simulink model "TB14_StageC_Regulated"  (R2025a)
settings: Solver=FixedStepDiscrete  StartTime=0  StopTime=TB.t_end  FixedStep=TB.dt  RelTol=1e-3
InitFcn:
  | % 모델과 같은 폴더의 초기화 스크립트를 실행해 P(설계 파라미터)와 TB(시험 조건)를 만든다.
  | run(fullfile(fileparts(get_param(bdroot, 'FileName')), 'TB14_init.m'));
values from neighbouring files (symbols this model uses):
  TB = struct()    [TB14_init.m]    (also in probe_TB14_solver.m = evalin('base', 'TB'); run_TB14.m = evalin('base', 'TB'))
libraries: fl_lib x59, nesl_utility x27
(part 1 of 2)
settings Model: Creator=hj000  LastModifiedBy=hj000
settings DataIOCC: SaveOutput=off  SignalLogging=off  SaveTime=off

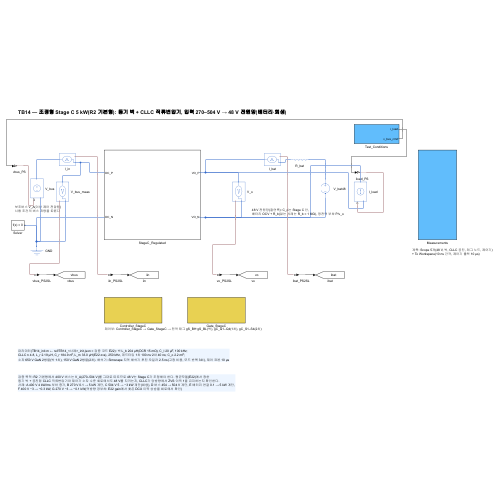
[thumbnail: Simulink's stored preview of the top-level diagram]
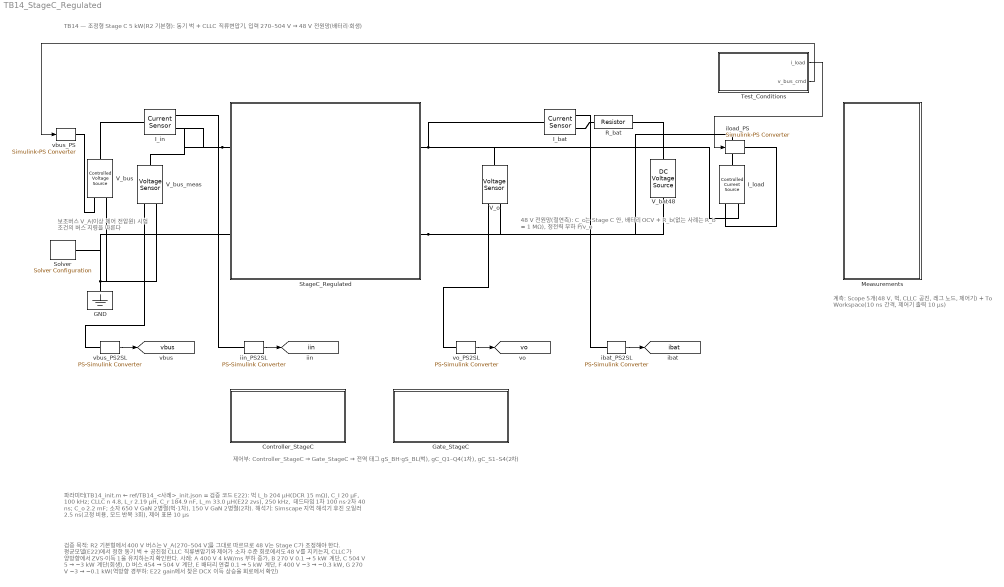
== system TB14_StageC_Regulated ==
  note: TB14 — 조정형 Stage C 5 kW(R2 기본형): 동기 벅 + CLLC 직류변압기, 입력 270–504 V → 48 V 전원망(배터리·회생)
  note: 보조버스 V_A(이상 제어 전압원)
      | 시험 조건의 버스 지령을 따른다
  note: 48 V 전원망(절연측): C_o는 Stage C 안,
      | 배터리 OCV + R_b(없는 사례는 R_b = 1 MΩ), 정전력 부하 P/v_o
  note: 제어부: Controller_StageC → Gate_StageC → 전역 태그 gS_BH·gS_BL(벅), gC_Q1–Q4(1차), gC_S1–S4(2차)
  note: 계측: Scope 5개(48 V, 벅, CLLC 공진, 레그 노드, 제어기)
      | + To Workspace(10 ns 간격, 제어기 출력 10 µs)
  note: 파라미터(TB14_init.m ← ref/TB14_<사례>_init.json = 검증 코드 E22): 벅 L_b 204 µH(DCR 15 mΩ), C_I 20 µF, 100 kHz;
      | CLLC n 4.8, L_r 2.19 µH, C_r 184.9 nF, L_m 33.0 µH(E22 zvs), 250 kHz, 데드타임 1차 100 ns·2차 40 ns; C_o 2.2 mF;
      | 소자 650 V GaN 2병렬(벅·1차), 150 V GaN 2병렬(2차). 해석기: Simscape 지역 해석기 후진 오일러 2.5 ns(고정 비용, 모드 반복 3회), 제어 표본 10 µs
  note: 검증 목적: R2 기본형에서 400 V 버스는 V_A(270–504 V)를 그대로 따르므로 48 V는 Stage C가 조정해야 한다. 평균모델(E22)에서 정한
      | 동기 벅 + 공진점 CLLC 직류변압기와 제어가 소자 수준 회로에서도 48 V를 지키는지, CLLC가 양방향에서 ZVS·이득 1을 유지하는지 확인한다.
      | 사례: A 400 V 4 kW/ms 부하 증가, B 270 V 0.1 → 5 kW 계단, C 504 V 5 → −3 kW 계단(회생), D 버스 454 → 504 V 계단, E 배터리 연결 0.1 → 5 kW 계단,
      | F 400 V −3 → −0.3 kW, G 270 V −3 → −0.1 kW(역방향 경부하: E22 gain에서 찾은 DCX 이득 상승을 회로에서 확인)
  Controller_StageC : Subsystem
  GND : fl_lib/Electrical/Electrical Elements/Electrical Reference
  Gate_StageC : Subsystem
  I_bat : fl_lib/Electrical/Electrical Sensors/Current Sensor
  I_in : fl_lib/Electrical/Electrical Sensors/Current Sensor
  I_load : fl_lib/Electrical/Electrical Sources/Controlled Current Source
  Measurements : Subsystem
  R_bat : fl_lib/Electrical/Electrical Elements/Resistor  R=TB.Rbat Ohm  i_specify=off  i_priority=None  i=0 A  i_nominal_specify=off  i_nominal_value=1  i_nominal_unit=A  v_specify=off  v_priority=None  v=0 V  v_nominal_specify=off  v_nominal_value=1  v_nominal_unit=V
  Solver : nesl_utility/Solver Configuration  PhysicalDomain=network_engine_domain  SubClassName=solver  LeftPortType=input  RightPortType=generic  Tones=[]  Harmonics=[]  SimulateNoise=off  Profile=off  UseLocalSampling=off  EnableSwitchedLinearOptims=on  FrequencyDomain=off  UseCCode=off  RelTol=0.001  AbsTol=0.001  MinStep=1e-09  ToWorkspace=off  RevertToSquareIcSolve=off  NumHomotopyIterations=100  PhasorMode=off  PhasorModeNumHarmonics=1  ConsistencySolver=NEWTON_XTOL_AFTER_FTOL  IndexReductionMethod=DerivativeReplacement  DoDC=off  ResidualTolerance=1e-9  ConsistencyTolSource=GLOBAL  ConsistencyAbsTol=0.001  ConsistencyRelTol=0.001  ConsistencyTolFactor=0.001  UseLocalSolver=on  LocalSolverChoice=NE_BACKWARD_EULER_ADVANCER  ResolveIndetEquations=on  FunctionEvalNumThread=1  LocalSolverSampleTime=TB.dt  DoFixedCost=on  MaxNonlinIter=3  MaxModeIter=2  ComputeImpulses=off  ImpulseIterations=2  LinearAlgebra=auto  LinearAlgebraNumThread=0  EquationFormulation=NE_TIME_EF  DelaysMemoryBudget=1024  AutomaticFiltering=on  FilteringTimeConstant=0.001  PartitionStorageMethod=AS_NEEDED  PartitionMemoryBudget=1024  PartitionMethod=ROBUST  MultibodyUseLocalSolver=off  MultibodyLocalSolverChoice=ODE1  MultibodyLocalSolverSampleTime=0.001
  StageC_Regulated : Subsystem
  Test_Conditions : Subsystem
  V_bat48 : fl_lib/Electrical/Electrical Sources/DC Voltage Source  v0=TB.OCV V
  V_bus : fl_lib/Electrical/Electrical Sources/Controlled Voltage Source
  V_bus_meas : fl_lib/Electrical/Electrical Sensors/Voltage Sensor
  V_o : fl_lib/Electrical/Electrical Sensors/Voltage Sensor
  ibat_PS2SL : nesl_utility/PS-Simulink Converter  PhysicalDomain=network_engine_domain  SubClassName=ps_output  LeftPortType=input  RightPortType=output  PseudoPeriodic=off  Frequencies=[]  VectorFormat=inherit  Unit=inherit  AffineConversion=off
  iin_PS2SL : nesl_utility/PS-Simulink Converter  PhysicalDomain=network_engine_domain  SubClassName=ps_output  LeftPortType=input  RightPortType=output  PseudoPeriodic=off  Frequencies=[]  VectorFormat=inherit  Unit=inherit  AffineConversion=off
  iload_PS : nesl_utility/Simulink-PS Converter  PhysicalDomain=network_engine_domain  SubClassName=ps_input  LeftPortType=input  RightPortType=output  PseudoPeriodic=off  Frequencies=[]  NoiseDistribution=none  NoiseParameters=[]  Unit=1  AffineConversion=off  FilteringAndDerivatives=provide  SimscapeFilterOrder=1  InputFilterTimeConstant=0.001  UdotUserProvided=0
  vbus_PS : nesl_utility/Simulink-PS Converter  PhysicalDomain=network_engine_domain  SubClassName=ps_input  LeftPortType=input  RightPortType=output  PseudoPeriodic=off  Frequencies=[]  NoiseDistribution=none  NoiseParameters=[]  Unit=1  AffineConversion=off  FilteringAndDerivatives=provide  SimscapeFilterOrder=1  InputFilterTimeConstant=0.001  UdotUserProvided=0
  vbus_PS2SL : nesl_utility/PS-Simulink Converter  PhysicalDomain=network_engine_domain  SubClassName=ps_output  LeftPortType=input  RightPortType=output  PseudoPeriodic=off  Frequencies=[]  VectorFormat=inherit  Unit=inherit  AffineConversion=off
  vo_PS2SL : nesl_utility/PS-Simulink Converter  PhysicalDomain=network_engine_domain  SubClassName=ps_output  LeftPortType=input  RightPortType=output  PseudoPeriodic=off  Frequencies=[]  VectorFormat=inherit  Unit=inherit  AffineConversion=off
  tag scope: ibat=global, iin=global, vbus=global, vo=global
  wires:
  vbus_PS2SL/1 -> [vbus]
  iin_PS2SL/1 -> [iin]
  vo_PS2SL/1 -> [vo]
  ibat_PS2SL/1 -> [ibat]
  Test_Conditions/1(i_load) -> iload_PS/1
  Test_Conditions/2(v_bus_cmd) -> vbus_PS/1
  connections:
  Solver/RConn1 -- V_bus/RConn2 -- StageC_Regulated/LConn2 -- GND/LConn1 -- V_bus_meas/RConn2
  vbus_PS/RConn1 -- V_bus/RConn1
  V_bus/LConn1 -- I_in/LConn1
  StageC_Regulated/LConn1 -- I_in/RConn2 -- V_bus_meas/LConn1
  V_o/LConn1 -- I_bat/LConn1 -- StageC_Regulated/RConn1 -- I_load/RConn2
  V_o/RConn2 -- V_bat48/RConn1 -- StageC_Regulated/RConn2 -- I_load/LConn1
  I_bat/RConn2 -- R_bat/LConn1
  R_bat/RConn1 -- V_bat48/LConn1
  iload_PS/RConn1 -- I_load/RConn1
  V_bus_meas/RConn1 -- vbus_PS2SL/LConn1
  I_in/RConn1 -- iin_PS2SL/LConn1
  V_o/RConn1 -- vo_PS2SL/LConn1
  I_bat/RConn1 -- ibat_PS2SL/LConn1

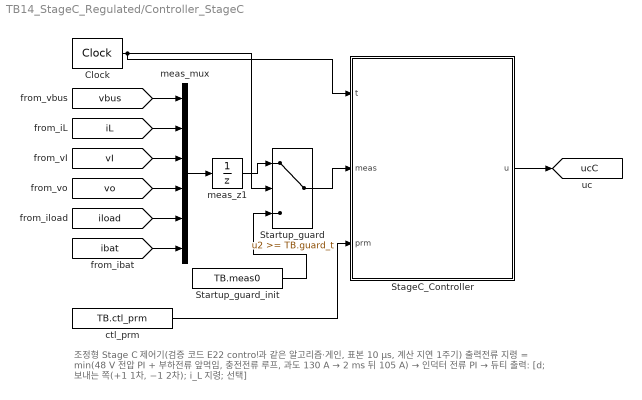
== system TB14_StageC_Regulated/Controller_StageC ==
  note: 조정형 Stage C 제어기(검증 코드 E22 control과 같은 알고리즘·게인, 표본 10 µs, 계산 지연 1주기)
      | 출력전류 지령 = min(48 V 전압 PI + 부하전류 앞먹임, 충전전류 루프, 과도 130 A → 2 ms 뒤 105 A) → 인덕터 전류 PI → 듀티
      | 출력: [d; 보내는 쪽(+1 1차, −1 2차); i_L 지령; 선택]
  Clock : DigitalClock  SampleTime=TB.dt
  StageC_Controller : MATLAB Function  TreatAsAtomicUnit=on
  Startup_guard : Switch  Threshold=TB.guard_t  SaturateOnIntegerOverflow=off  InputSameDT=off
  Startup_guard_init : Constant  Value=TB.meas0
  ctl_prm : Constant  Value=TB.ctl_prm
  meas_mux : Mux  Inputs=6
  meas_z1 : UnitDelay  InitialCondition=TB.meas0  SampleTime=TB.dt  HasFrameUpgradeWarning=on
  tag scope: ucC=global
  wires:
  [vbus] -> meas_mux/1
  [iL] -> meas_mux/2
  [vI] -> meas_mux/3
  [vo] -> meas_mux/4
  [iload] -> meas_mux/5
  [ibat] -> meas_mux/6
  meas_mux/1 -> meas_z1/1
  Startup_guard_init/1 -> Startup_guard/3
  meas_z1/1 -> Startup_guard/1
  Clock/1 -> Startup_guard/2, StageC_Controller/1(t)
  Startup_guard/1 -> StageC_Controller/2(meas)
  ctl_prm/1 -> StageC_Controller/3(prm)
  StageC_Controller/1(u) -> [ucC]

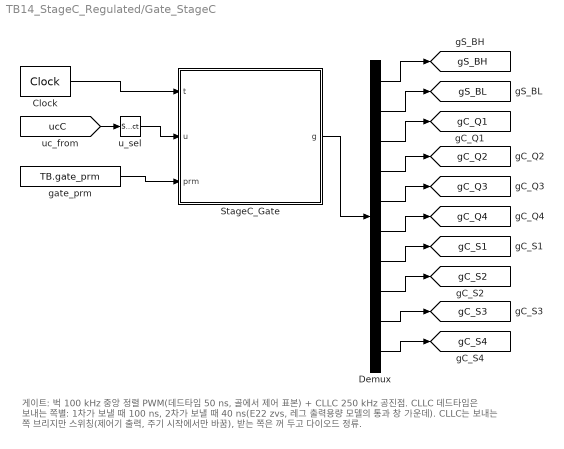
== system TB14_StageC_Regulated/Gate_StageC ==
  note: 게이트: 벅 100 kHz 중앙 정렬 PWM(데드타임 50 ns, 골에서 제어 표본) + CLLC 250 kHz 공진점.
      | CLLC 데드타임은 보내는 쪽별: 1차가 보낼 때 100 ns, 2차가 보낼 때 40 ns(E22 zvs, 레그 출력용량 모델의 통과 창 가운데).
      | CLLC는 보내는 쪽 브리지만 스위칭(제어기 출력, 주기 시작에서만 바꿈), 받는 쪽은 꺼 두고 다이오드 정류.
  Clock : DigitalClock  SampleTime=TB.dt
  Demux : Demux  Outputs=10
  StageC_Gate : MATLAB Function  TreatAsAtomicUnit=on
  gate_prm : Constant  Value=TB.gate_prm
  u_sel : Selector  InputPortWidth=4  IndexOptions=Index vector (dialog)  Indices=[1 2]  OutputSizes=1
  tag scope: gC_Q1=global, gC_Q2=global, gC_Q3=global, gC_Q4=global, gC_S1=global, gC_S2=global, gC_S3=global, gC_S4=global, gS_BH=global, gS_BL=global
  wires:
  [ucC] -> u_sel/1
  Clock/1 -> StageC_Gate/1(t)
  u_sel/1 -> StageC_Gate/2(u)
  gate_prm/1 -> StageC_Gate/3(prm)
  StageC_Gate/1(g) -> Demux/1
  Demux/1 -> [gS_BH]
  Demux/2 -> [gS_BL]
  Demux/3 -> [gC_Q1]
  Demux/4 -> [gC_Q2]
  Demux/5 -> [gC_Q3]
  Demux/6 -> [gC_Q4]
  Demux/7 -> [gC_S1]
  Demux/8 -> [gC_S2]
  Demux/9 -> [gC_S3]
  Demux/10 -> [gC_S4]

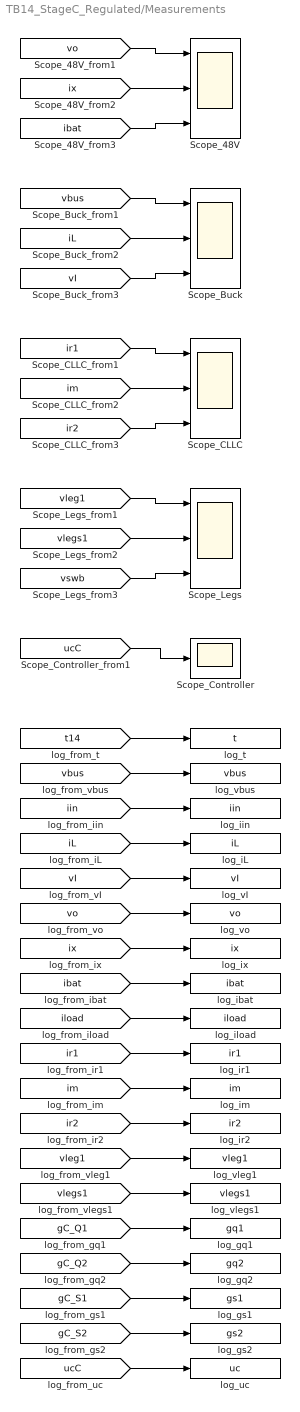
== system TB14_StageC_Regulated/Measurements ==
  Scope_48V : Scope  NumInputPorts=3
      settings: Title=Scope 48V
  Scope_Buck : Scope  NumInputPorts=3
      settings: Title=Scope Buck
  Scope_CLLC : Scope  NumInputPorts=3
      settings: Title=Scope CLLC
  Scope_Controller : Scope
      settings: Title=Scope Controller
  Scope_Legs : Scope  NumInputPorts=3
      settings: Title=Scope Legs
  log_gq1 : ToWorkspace  VariableName=gq1  SampleTime=-1
      settings: Decimation=4
  log_gq2 : ToWorkspace  VariableName=gq2  SampleTime=-1
      settings: Decimation=4
  log_gs1 : ToWorkspace  VariableName=gs1  SampleTime=-1
      settings: Decimation=4
  log_gs2 : ToWorkspace  VariableName=gs2  SampleTime=-1
      settings: Decimation=4
  log_iL : ToWorkspace  VariableName=iL  SampleTime=-1
      settings: Decimation=4
  log_ibat : ToWorkspace  VariableName=ibat  SampleTime=-1
      settings: Decimation=4
  log_iin : ToWorkspace  VariableName=iin  SampleTime=-1
      settings: Decimation=4
  log_iload : ToWorkspace  VariableName=iload  SampleTime=-1
      settings: Decimation=4
  log_im : ToWorkspace  VariableName=im  SampleTime=-1
      settings: Decimation=4
  log_ir1 : ToWorkspace  VariableName=ir1  SampleTime=-1
      settings: Decimation=4
  log_ir2 : ToWorkspace  VariableName=ir2  SampleTime=-1
      settings: Decimation=4
  log_ix : ToWorkspace  VariableName=ix  SampleTime=-1
      settings: Decimation=4
  log_t : ToWorkspace  VariableName=t  SampleTime=-1
      settings: Decimation=4
  log_uc : ToWorkspace  VariableName=uc  SampleTime=-1
      settings: Decimation=4000
  log_vI : ToWorkspace  VariableName=vI  SampleTime=-1
      settings: Decimation=4
  log_vbus : ToWorkspace  VariableName=vbus  SampleTime=-1
      settings: Decimation=4
  log_vleg1 : ToWorkspace  VariableName=vleg1  SampleTime=-1
      settings: Decimation=4
  log_vlegs1 : ToWorkspace  VariableName=vlegs1  SampleTime=-1
      settings: Decimation=4
  log_vo : ToWorkspace  VariableName=vo  SampleTime=-1
      settings: Decimation=4
  wires:
  [vo] -> Scope_48V/1
  [ix] -> Scope_48V/2
  [ibat] -> Scope_48V/3
  [vbus] -> Scope_Buck/1
  [iL] -> Scope_Buck/2
  [vI] -> Scope_Buck/3
  [ir1] -> Scope_CLLC/1
  [im] -> Scope_CLLC/2
  [ir2] -> Scope_CLLC/3
  [vleg1] -> Scope_Legs/1
  [vlegs1] -> Scope_Legs/2
  [vswb] -> Scope_Legs/3
  [ucC] -> Scope_Controller/1
  [t14] -> log_t/1
  [vbus] -> log_vbus/1
  [iin] -> log_iin/1
  [iL] -> log_iL/1
  [vI] -> log_vI/1
  [vo] -> log_vo/1
  [ix] -> log_ix/1
  [ibat] -> log_ibat/1
  [iload] -> log_iload/1
  [ir1] -> log_ir1/1
  [im] -> log_im/1
  [ir2] -> log_ir2/1
  [vleg1] -> log_vleg1/1
  [vlegs1] -> log_vlegs1/1
  [gC_Q1] -> log_gq1/1
  [gC_Q2] -> log_gq2/1
  [gC_S1] -> log_gs1/1
  [gC_S2] -> log_gs2/1
  [ucC] -> log_uc/1

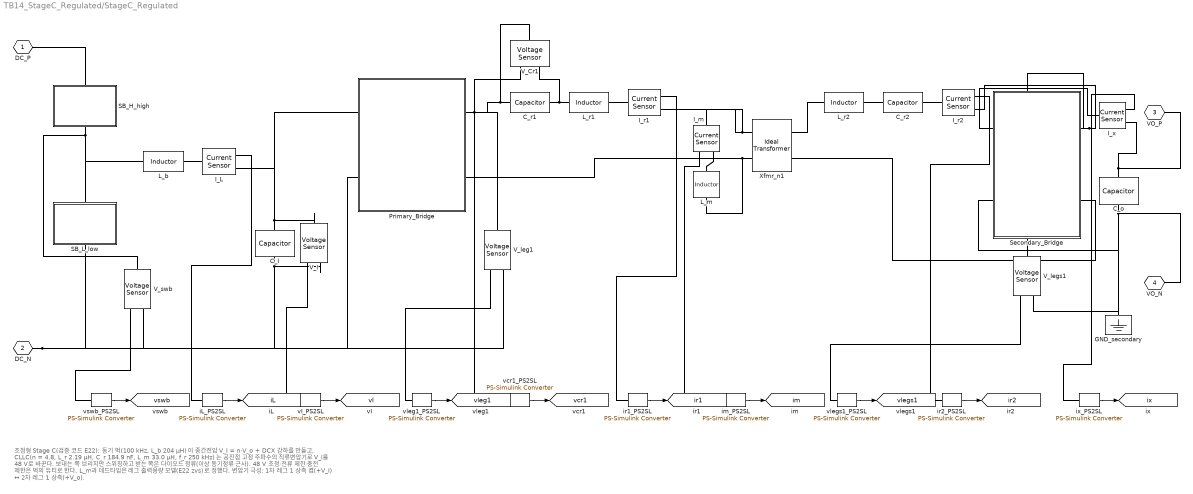
== system TB14_StageC_Regulated/StageC_Regulated ==
  note: 조정형 Stage C(검증 코드 E22): 동기 벅(100 kHz, L_b 204 µH)이 중간전압 V_I = n·V_o + DCX 강하를 만들고,
      | CLLC(n = 4.8, L_r 2.19 µH, C_r 184.9 nF, L_m 33.0 µH, f_r 250 kHz)는 공진점 고정 주파수의 직류변압기로 V_I를 48 V로 바꾼다.
      | 보내는 쪽 브리지만 스위칭하고 받는 쪽은 다이오드 정류(이상 동기정류 근사). 48 V 조정·전류 제한·충전 제한은 벅의 듀티로 한다.
      | L_m과 데드타임은 레그 출력용량 모델(E22 zvs)로 정했다. 변압기 극성: 1차 레그 1 상측 켬(+V_I) ↔ 2차 레그 1 상측(+V_o).
  C_I : fl_lib/Electrical/Electrical Elements/Capacitor  c=TB.C.CI F  r=1e-6 Ohm  g=0 1/Ohm  i_specify=off  i_priority=None  i=0 A  i_nominal_specify=off  i_nominal_value=1  i_nominal_unit=A  v_specify=off  v_priority=None  v=0 V  v_nominal_specify=off  v_nominal_value=1  v_nominal_unit=V  vc_specify=on  vc_priority=High  vc=TB.x0(2) V  vc_nominal_specify=off  vc_nominal_value=1  vc_nominal_unit=V
  C_o : fl_lib/Electrical/Electrical Elements/Capacitor  c=TB.C.Co F  r=1e-6 Ohm  g=0 1/Ohm  i_specify=off  i_priority=None  i=0 A  i_nominal_specify=off  i_nominal_value=1  i_nominal_unit=A  v_specify=off  v_priority=None  v=0 V  v_nominal_specify=off  v_nominal_value=1  v_nominal_unit=V  vc_specify=on  vc_priority=High  vc=TB.x0(3) V  vc_nominal_specify=off  vc_nominal_value=1  vc_nominal_unit=V
  C_r1 : fl_lib/Electrical/Electrical Elements/Capacitor  c=TB.C.Cr1 F  r=1e-6 Ohm  g=0 1/Ohm  i_specify=off  i_priority=None  i=0 A  i_nominal_specify=off  i_nominal_value=1  i_nominal_unit=A  v_specify=off  v_priority=None  v=0 V  v_nominal_specify=off  v_nominal_value=1  v_nominal_unit=V  vc_specify=on  vc_priority=High  vc=0 V  vc_nominal_specify=off  vc_nominal_value=1  vc_nominal_unit=V
  C_r2 : fl_lib/Electrical/Electrical Elements/Capacitor  c=TB.C.Cr2 F  r=1e-6 Ohm  g=0 1/Ohm  i_specify=off  i_priority=None  i=0 A  i_nominal_specify=off  i_nominal_value=1  i_nominal_unit=A  v_specify=off  v_priority=None  v=0 V  v_nominal_specify=off  v_nominal_value=1  v_nominal_unit=V  vc_specify=on  vc_priority=High  vc=0 V  vc_nominal_specify=off  vc_nominal_value=1  vc_nominal_unit=V
  GND_secondary : fl_lib/Electrical/Electrical Elements/Electrical Reference
  I_L : fl_lib/Electrical/Electrical Sensors/Current Sensor
  I_m : fl_lib/Electrical/Electrical Sensors/Current Sensor
  I_r1 : fl_lib/Electrical/Electrical Sensors/Current Sensor
  I_r2 : fl_lib/Electrical/Electrical Sensors/Current Sensor
  I_x : fl_lib/Electrical/Electrical Sensors/Current Sensor
  L_b : fl_lib/Electrical/Electrical Elements/Inductor  l=TB.C.L H  r=TB.C.RL Ohm  g=1e-9 1/Ohm  i_specify=off  i_priority=None  i=0 A  i_nominal_specify=off  i_nominal_value=1  i_nominal_unit=A  v_specify=off  v_priority=None  v=0 V  v_nominal_specify=off  v_nominal_value=1  v_nominal_unit=V  i_L_specify=on  i_L_priority=High  i_L=TB.x0(1) A  i_L_nominal_specify=off  i_L_nominal_value=1  i_L_nominal_unit=A
  L_m : fl_lib/Electrical/Electrical Elements/Inductor  l=TB.C.Lm H  r=0 Ohm  g=1e-9 1/Ohm  i_specify=off  i_priority=None  i=0 A  i_nominal_specify=off  i_nominal_value=1  i_nominal_unit=A  v_specify=off  v_priority=None  v=0 V  v_nominal_specify=off  v_nominal_value=1  v_nominal_unit=V  i_L_specify=on  i_L_priority=High  i_L=0 A  i_L_nominal_specify=off  i_L_nominal_value=1  i_L_nominal_unit=A
  L_r1 : fl_lib/Electrical/Electrical Elements/Inductor  l=TB.C.Lr1 H  r=TB.C.Rw1 Ohm  g=1e-9 1/Ohm  i_specify=off  i_priority=None  i=0 A  i_nominal_specify=off  i_nominal_value=1  i_nominal_unit=A  v_specify=off  v_priority=None  v=0 V  v_nominal_specify=off  v_nominal_value=1  v_nominal_unit=V  i_L_specify=on  i_L_priority=High  i_L=0 A  i_L_nominal_specify=off  i_L_nominal_value=1  i_L_nominal_unit=A
  L_r2 : fl_lib/Electrical/Electrical Elements/Inductor  l=TB.C.Lr2 H  r=TB.C.Rw2 Ohm  g=1e-9 1/Ohm  i_specify=off  i_priority=None  i=0 A  i_nominal_specify=off  i_nominal_value=1  i_nominal_unit=A  v_specify=off  v_priority=None  v=0 V  v_nominal_specify=off  v_nominal_value=1  v_nominal_unit=V  i_L_specify=on  i_L_priority=High  i_L=0 A  i_L_nominal_specify=off  i_L_nominal_value=1  i_L_nominal_unit=A
  Primary_Bridge : Subsystem
  SB_H_high : Subsystem  mask(PRISM-Hub switch cell){Ron=TB.SB.Ron, Goff=TB.SB.Goff, Vf=TB.SB.Vf, Rd=TB.SB.Rd, Goffd=TB.SB.Goffd, Coss=TB.SB.Coss}
      mask prompts: Ron "도통 저항 R_on [Ohm]"; Goff "차단 컨덕턴스 G_off [S]"; Vf "다이오드 순방향 전압 Vf [V]"; Rd "다이오드 도통 저항 R_d [Ohm]"; Goffd "다이오드 차단 컨덕턴스 [S]"; Coss "출력용량 C_oss [F]"
      mask help: 전력 반도체 스위치 셀 SB_H. 게이트 태그 gS_BH.
      settings: AttributesFormatString=gate: gS_BH
      mask Display:
      | plot([0.50 0.50 ],[0.95 0.65 ],[0.50 0.74 ],[0.65 0.35 ],[0.50 0.50 ],[0.35 0.05 ]);
      | plot([0.50 0.20 0.20 ],[0.80 0.80 0.58 ],[0.20 0.20 0.50 ],[0.42 0.20 0.20 ]);
      | plot([0.20 0.10 0.30 0.20 ],[0.58 0.42 0.42 0.58 ],[0.10 0.30 ],[0.58 0.58 ]);
      | port_label('LConn',1,'D');
      | port_label('RConn',1,'S');
  SB_L_low : Subsystem  mask(PRISM-Hub switch cell){Ron=TB.SB.Ron, Goff=TB.SB.Goff, Vf=TB.SB.Vf, Rd=TB.SB.Rd, Goffd=TB.SB.Goffd, Coss=TB.SB.Coss}
      mask prompts: Ron "도통 저항 R_on [Ohm]"; Goff "차단 컨덕턴스 G_off [S]"; Vf "다이오드 순방향 전압 Vf [V]"; Rd "다이오드 도통 저항 R_d [Ohm]"; Goffd "다이오드 차단 컨덕턴스 [S]"; Coss "출력용량 C_oss [F]"
      mask help: 전력 반도체 스위치 셀 SB_L. 게이트 태그 gS_BL.
      settings: AttributesFormatString=gate: gS_BL
      mask Display:
      | plot([0.50 0.50 ],[0.95 0.65 ],[0.50 0.74 ],[0.65 0.35 ],[0.50 0.50 ],[0.35 0.05 ]);
      | plot([0.50 0.20 0.20 ],[0.80 0.80 0.58 ],[0.20 0.20 0.50 ],[0.42 0.20 0.20 ]);
      | plot([0.20 0.10 0.30 0.20 ],[0.58 0.42 0.42 0.58 ],[0.10 0.30 ],[0.58 0.58 ]);
      | port_label('LConn',1,'D');
      | port_label('RConn',1,'S');
  Secondary_Bridge : Subsystem
  V_Cr1 : fl_lib/Electrical/Electrical Sensors/Voltage Sensor
  V_I : fl_lib/Electrical/Electrical Sensors/Voltage Sensor
  V_leg1 : fl_lib/Electrical/Electrical Sensors/Voltage Sensor
  V_legs1 : fl_lib/Electrical/Electrical Sensors/Voltage Sensor
  V_swb : fl_lib/Electrical/Electrical Sensors/Voltage Sensor
  Xfmr_n1 : fl_lib/Electrical/Electrical Elements/Ideal Transformer  n=TB.C.n  i1_specify=off  i1_priority=None  i1=0 A  i1_nominal_specify=off  i1_nominal_value=1  i1_nominal_unit=A  v1_specify=off  v1_priority=None  v1=0 V  v1_nominal_specify=off  v1_nominal_value=1  v1_nominal_unit=V  i2_specify=off  i2_priority=None  i2=0 A  i2_nominal_specify=off  i2_nominal_value=1  i2_nominal_unit=A  v2_specify=off  v2_priority=None  v2=0 V  v2_nominal_specify=off  v2_nominal_value=1  v2_nominal_unit=V
  iL_PS2SL : nesl_utility/PS-Simulink Converter  PhysicalDomain=network_engine_domain  SubClassName=ps_output  LeftPortType=input  RightPortType=output  PseudoPeriodic=off  Frequencies=[]  VectorFormat=inherit  Unit=inherit  AffineConversion=off
  im_PS2SL : nesl_utility/PS-Simulink Converter  PhysicalDomain=network_engine_domain  SubClassName=ps_output  LeftPortType=input  RightPortType=output  PseudoPeriodic=off  Frequencies=[]  VectorFormat=inherit  Unit=inherit  AffineConversion=off
  ir1_PS2SL : nesl_utility/PS-Simulink Converter  PhysicalDomain=network_engine_domain  SubClassName=ps_output  LeftPortType=input  RightPortType=output  PseudoPeriodic=off  Frequencies=[]  VectorFormat=inherit  Unit=inherit  AffineConversion=off
  ir2_PS2SL : nesl_utility/PS-Simulink Converter  PhysicalDomain=network_engine_domain  SubClassName=ps_output  LeftPortType=input  RightPortType=output  PseudoPeriodic=off  Frequencies=[]  VectorFormat=inherit  Unit=inherit  AffineConversion=off
  ix_PS2SL : nesl_utility/PS-Simulink Converter  PhysicalDomain=network_engine_domain  SubClassName=ps_output  LeftPortType=input  RightPortType=output  PseudoPeriodic=off  Frequencies=[]  VectorFormat=inherit  Unit=inherit  AffineConversion=off
  vI_PS2SL : nesl_utility/PS-Simulink Converter  PhysicalDomain=network_engine_domain  SubClassName=ps_output  LeftPortType=input  RightPortType=output  PseudoPeriodic=off  Frequencies=[]  VectorFormat=inherit  Unit=inherit  AffineConversion=off
  vcr1_PS2SL : nesl_utility/PS-Simulink Converter  PhysicalDomain=network_engine_domain  SubClassName=ps_output  LeftPortType=input  RightPortType=output  PseudoPeriodic=off  Frequencies=[]  VectorFormat=inherit  Unit=inherit  AffineConversion=off
  vleg1_PS2SL : nesl_utility/PS-Simulink Converter  PhysicalDomain=network_engine_domain  SubClassName=ps_output  LeftPortType=input  RightPortType=output  PseudoPeriodic=off  Frequencies=[]  VectorFormat=inherit  Unit=inherit  AffineConversion=off
  vlegs1_PS2SL : nesl_utility/PS-Simulink Converter  PhysicalDomain=network_engine_domain  SubClassName=ps_output  LeftPortType=input  RightPortType=output  PseudoPeriodic=off  Frequencies=[]  VectorFormat=inherit  Unit=inherit  AffineConversion=off
  vswb_PS2SL : nesl_utility/PS-Simulink Converter  PhysicalDomain=network_engine_domain  SubClassName=ps_output  LeftPortType=input  RightPortType=output  PseudoPeriodic=off  Frequencies=[]  VectorFormat=inherit  Unit=inherit  AffineConversion=off
  DC_P : PMIOPort  Side=Left
  DC_N : PMIOPort  Port=2  Side=Left
  VO_P : PMIOPort  Port=3  Side=Right
  VO_N : PMIOPort  Port=4  Side=Right
  tag scope: iL=global, im=global, ir1=global, ir2=global, ix=global, vI=global, vcr1=global, vleg1=global, vlegs1=global, vswb=global
  wires:
  iL_PS2SL/1 -> [iL]
  vI_PS2SL/1 -> [vI]
  vswb_PS2SL/1 -> [vswb]
  ir1_PS2SL/1 -> [ir1]
  im_PS2SL/1 -> [im]
  ir2_PS2SL/1 -> [ir2]
  ix_PS2SL/1 -> [ix]
  vcr1_PS2SL/1 -> [vcr1]
  vleg1_PS2SL/1 -> [vleg1]
  vlegs1_PS2SL/1 -> [vlegs1]
  connections:
  SB_H_high/LConn1 -- DC_P/RConn1
  SB_L_low/LConn1 -- SB_H_high/RConn1 -- L_b/LConn1 -- V_swb/LConn1
  SB_L_low/RConn1 -- C_I/RConn1 -- V_I/RConn2 -- V_swb/RConn2 -- Primary_Bridge/LConn2 -- DC_N/RConn1 -- V_leg1/RConn2
  L_b/RConn1 -- I_L/LConn1
  I_L/RConn2 -- V_I/LConn1 -- C_I/LConn1 -- Primary_Bridge/LConn1
  C_r1/LConn1 -- Primary_Bridge/RConn1 -- V_leg1/LConn1 -- V_Cr1/LConn1
  L_r1/LConn1 -- C_r1/RConn1 -- V_Cr1/RConn2
  L_r1/RConn1 -- I_r1/LConn1
  Xfmr_n1/LConn1 -- I_r1/RConn2 -- I_m/LConn1
  Primary_Bridge/RConn2 -- Xfmr_n1/LConn2 -- L_m/RConn1
  I_m/RConn2 -- L_m/LConn1
  Xfmr_n1/RConn1 -- L_r2/LConn1
  L_r2/RConn1 -- C_r2/LConn1
  C_r2/RConn1 -- I_r2/LConn1
  Secondary_Bridge/RConn1 -- I_r2/RConn2 -- V_legs1/LConn1
  Xfmr_n1/RConn2 -- Secondary_Bridge/RConn2
  Secondary_Bridge/LConn1 -- I_x/LConn1
  C_o/LConn1 -- I_x/RConn2 -- VO_P/RConn1
  Secondary_Bridge/LConn2 -- VO_N/RConn1 -- V_legs1/RConn2 -- C_o/RConn1 -- GND_secondary/LConn1
  I_L/RConn1 -- iL_PS2SL/LConn1
  V_I/RConn1 -- vI_PS2SL/LConn1
  V_swb/RConn1 -- vswb_PS2SL/LConn1
  I_r1/RConn1 -- ir1_PS2SL/LConn1
  I_m/RConn1 -- im_PS2SL/LConn1
  I_r2/RConn1 -- ir2_PS2SL/LConn1
  I_x/RConn1 -- ix_PS2SL/LConn1
  V_Cr1/RConn1 -- vcr1_PS2SL/LConn1
  V_leg1/RConn1 -- vleg1_PS2SL/LConn1
  V_legs1/RConn1 -- vlegs1_PS2SL/LConn1

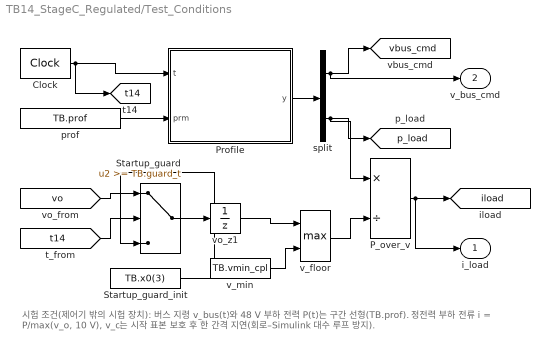
== system TB14_StageC_Regulated/Test_Conditions ==
  note: 시험 조건(제어기 밖의 시험 장치): 버스 지령 v_bus(t)와 48 V 부하 전력 P(t)는 구간 선형(TB.prof).
      | 정전력 부하 전류 i = P/max(v_o, 10 V), v_o는 시작 표본 보호 후 한 간격 지연(회로–Simulink 대수 루프 방지).
  Clock : DigitalClock  SampleTime=TB.dt
  P_over_v : Product  Inputs=*/
  Profile : MATLAB Function  TreatAsAtomicUnit=on
  Startup_guard : Switch  Threshold=TB.guard_t  SaturateOnIntegerOverflow=off  InputSameDT=off
  Startup_guard_init : Constant  Value=TB.x0(3)
  prof : Constant  Value=TB.prof
  split : Demux  Outputs=2
  v_floor : MinMax  Function=max  Inputs=2
  v_min : Constant  Value=TB.vmin_cpl
  vo_z1 : UnitDelay  SampleTime=TB.dt  HasFrameUpgradeWarning=on
  i_load : Outport
  v_bus_cmd : Outport  Port=2
  tag scope: iload=global, p_load=global, t14=global, vbus_cmd=global
  wires:
  Clock/1 -> Profile/1(t), [t14]
  prof/1 -> Profile/2(prm)
  Profile/1(y) -> split/1
  split/1 -> [vbus_cmd], v_bus_cmd/1
  split/2 -> [p_load], P_over_v/1
  Startup_guard_init/1 -> Startup_guard/3
  [vo] -> Startup_guard/1
  [t14] -> Startup_guard/2
  Startup_guard/1 -> vo_z1/1
  vo_z1/1 -> v_floor/1
  v_min/1 -> v_floor/2
  v_floor/1 -> P_over_v/2
  P_over_v/1 -> [iload], i_load/1

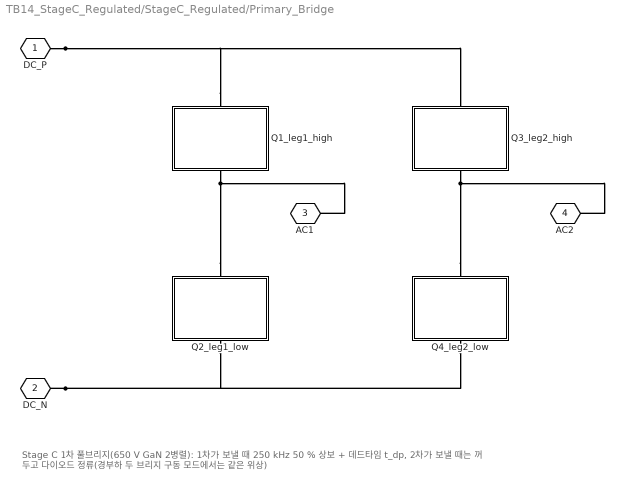
== system TB14_StageC_Regulated/StageC_Regulated/Primary_Bridge ==
  note: Stage C 1차 풀브리지(650 V GaN 2병렬): 1차가 보낼 때 250 kHz 50 % 상보 + 데드타임 t_dp, 2차가 보낼 때는 꺼 두고 다이오드 정류(경부하 두 브리지 구동 모드에서는 같은 위상)
  Q1_leg1_high : Subsystem  mask(PRISM-Hub switch cell){Ron=TB.CP.Ron, Goff=TB.CP.Goff, Vf=TB.CP.Vf, Rd=TB.CP.Rd, Goffd=TB.CP.Goffd, Coss=TB.CP.Coss}
      mask prompts: Ron "도통 저항 R_on [Ohm]"; Goff "차단 컨덕턴스 G_off [S]"; Vf "다이오드 순방향 전압 Vf [V]"; Rd "다이오드 도통 저항 R_d [Ohm]"; Goffd "다이오드 차단 컨덕턴스 [S]"; Coss "출력용량 C_oss [F]"
      mask help: 전력 반도체 스위치 셀 Q1_leg1_high. 게이트 태그 gC_Q1.
      settings: AttributesFormatString=gate: gC_Q1
      mask Display:
      | plot([0.50 0.50 ],[0.95 0.65 ],[0.50 0.74 ],[0.65 0.35 ],[0.50 0.50 ],[0.35 0.05 ]);
      | plot([0.50 0.20 0.20 ],[0.80 0.80 0.58 ],[0.20 0.20 0.50 ],[0.42 0.20 0.20 ]);
      | plot([0.20 0.10 0.30 0.20 ],[0.58 0.42 0.42 0.58 ],[0.10 0.30 ],[0.58 0.58 ]);
      | port_label('LConn',1,'D');
      | port_label('RConn',1,'S');
  Q2_leg1_low : Subsystem  mask(PRISM-Hub switch cell){Ron=TB.CP.Ron, Goff=TB.CP.Goff, Vf=TB.CP.Vf, Rd=TB.CP.Rd, Goffd=TB.CP.Goffd, Coss=TB.CP.Coss}
      mask prompts: Ron "도통 저항 R_on [Ohm]"; Goff "차단 컨덕턴스 G_off [S]"; Vf "다이오드 순방향 전압 Vf [V]"; Rd "다이오드 도통 저항 R_d [Ohm]"; Goffd "다이오드 차단 컨덕턴스 [S]"; Coss "출력용량 C_oss [F]"
      mask help: 전력 반도체 스위치 셀 Q2_leg1_low. 게이트 태그 gC_Q2.
      settings: AttributesFormatString=gate: gC_Q2
      mask Display:
      | plot([0.50 0.50 ],[0.95 0.65 ],[0.50 0.74 ],[0.65 0.35 ],[0.50 0.50 ],[0.35 0.05 ]);
      | plot([0.50 0.20 0.20 ],[0.80 0.80 0.58 ],[0.20 0.20 0.50 ],[0.42 0.20 0.20 ]);
      | plot([0.20 0.10 0.30 0.20 ],[0.58 0.42 0.42 0.58 ],[0.10 0.30 ],[0.58 0.58 ]);
      | port_label('LConn',1,'D');
      | port_label('RConn',1,'S');
  Q3_leg2_high : Subsystem  mask(PRISM-Hub switch cell){Ron=TB.CP.Ron, Goff=TB.CP.Goff, Vf=TB.CP.Vf, Rd=TB.CP.Rd, Goffd=TB.CP.Goffd, Coss=TB.CP.Coss}
      mask prompts: Ron "도통 저항 R_on [Ohm]"; Goff "차단 컨덕턴스 G_off [S]"; Vf "다이오드 순방향 전압 Vf [V]"; Rd "다이오드 도통 저항 R_d [Ohm]"; Goffd "다이오드 차단 컨덕턴스 [S]"; Coss "출력용량 C_oss [F]"
      mask help: 전력 반도체 스위치 셀 Q3_leg2_high. 게이트 태그 gC_Q3.
      settings: AttributesFormatString=gate: gC_Q3
      mask Display:
      | plot([0.50 0.50 ],[0.95 0.65 ],[0.50 0.74 ],[0.65 0.35 ],[0.50 0.50 ],[0.35 0.05 ]);
      | plot([0.50 0.20 0.20 ],[0.80 0.80 0.58 ],[0.20 0.20 0.50 ],[0.42 0.20 0.20 ]);
      | plot([0.20 0.10 0.30 0.20 ],[0.58 0.42 0.42 0.58 ],[0.10 0.30 ],[0.58 0.58 ]);
      | port_label('LConn',1,'D');
      | port_label('RConn',1,'S');
  Q4_leg2_low : Subsystem  mask(PRISM-Hub switch cell){Ron=TB.CP.Ron, Goff=TB.CP.Goff, Vf=TB.CP.Vf, Rd=TB.CP.Rd, Goffd=TB.CP.Goffd, Coss=TB.CP.Coss}
      mask prompts: Ron "도통 저항 R_on [Ohm]"; Goff "차단 컨덕턴스 G_off [S]"; Vf "다이오드 순방향 전압 Vf [V]"; Rd "다이오드 도통 저항 R_d [Ohm]"; Goffd "다이오드 차단 컨덕턴스 [S]"; Coss "출력용량 C_oss [F]"
      mask help: 전력 반도체 스위치 셀 Q4_leg2_low. 게이트 태그 gC_Q4.
      settings: AttributesFormatString=gate: gC_Q4
      mask Display:
      | plot([0.50 0.50 ],[0.95 0.65 ],[0.50 0.74 ],[0.65 0.35 ],[0.50 0.50 ],[0.35 0.05 ]);
      | plot([0.50 0.20 0.20 ],[0.80 0.80 0.58 ],[0.20 0.20 0.50 ],[0.42 0.20 0.20 ]);
      | plot([0.20 0.10 0.30 0.20 ],[0.58 0.42 0.42 0.58 ],[0.10 0.30 ],[0.58 0.58 ]);
      | port_label('LConn',1,'D');
      | port_label('RConn',1,'S');
  DC_P : PMIOPort  Side=Left
  DC_N : PMIOPort  Port=2  Side=Left
  AC1 : PMIOPort  Port=3  Side=Right
  AC2 : PMIOPort  Port=4  Side=Right
  connections:
  Q1_leg1_high/LConn1 -- DC_P/RConn1 -- Q3_leg2_high/LConn1
  Q2_leg1_low/LConn1 -- Q1_leg1_high/RConn1 -- AC1/RConn1
  Q4_leg2_low/LConn1 -- Q3_leg2_high/RConn1 -- AC2/RConn1
  DC_N/RConn1 -- Q2_leg1_low/RConn1 -- Q4_leg2_low/RConn1

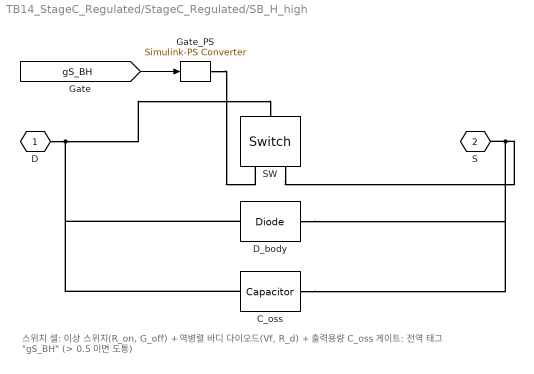
== system TB14_StageC_Regulated/StageC_Regulated/SB_H_high ==
  note: 스위치 셀: 이상 스위치(R_on, G_off) + 역병렬 바디 다이오드(Vf, R_d) + 출력용량 C_oss
      | 게이트: 전역 태그 "gS_BH" (> 0.5 이면 도통)
  C_oss : fl_lib/Electrical/Electrical Elements/Capacitor  c=Coss F  r=1e-6 Ohm  g=0 1/Ohm  i_specify=off  i_priority=None  i=0 A  i_nominal_specify=off  i_nominal_value=1  i_nominal_unit=A  v_specify=off  v_priority=None  v=0 V  v_nominal_specify=off  v_nominal_value=1  v_nominal_unit=V  vc_specify=off  vc_priority=High  vc=0 V  vc_nominal_specify=off  vc_nominal_value=1  vc_nominal_unit=V
  D_body : fl_lib/Electrical/Electrical Elements/Diode  Vf=Vf V  Ron=Rd Ohm  Goff=Goffd 1/Ohm  i_specify=off  i_priority=None  i=0 A  i_nominal_specify=off  i_nominal_value=1  i_nominal_unit=A  v_specify=off  v_priority=None  v=0 V  v_nominal_specify=off  v_nominal_value=1  v_nominal_unit=V
  Gate_PS : nesl_utility/Simulink-PS Converter  PhysicalDomain=network_engine_domain  SubClassName=ps_input  LeftPortType=input  RightPortType=output  PseudoPeriodic=off  Frequencies=[]  NoiseDistribution=none  NoiseParameters=[]  Unit=1  AffineConversion=off  FilteringAndDerivatives=zero  SimscapeFilterOrder=1  InputFilterTimeConstant=0.001  UdotUserProvided=0
  SW : fl_lib/Electrical/Electrical Elements/Switch  R_closed=Ron Ohm  G_open=Goff 1/Ohm  Threshold=0.5  i_specify=off  i_priority=None  i=0 A  i_nominal_specify=off  i_nominal_value=1  i_nominal_unit=A  v_specify=off  v_priority=None  v=0 V  v_nominal_specify=off  v_nominal_value=1  v_nominal_unit=V
  D : PMIOPort  Side=Left
  S : PMIOPort  Port=2  Side=Right
  wires:
  [gS_BH] -> Gate_PS/1
  connections:
  Gate_PS/RConn1 -- SW/RConn1
  SW/LConn1 -- D/RConn1 -- D_body/RConn1 -- C_oss/LConn1
  SW/RConn2 -- D_body/LConn1 -- S/RConn1 -- C_oss/RConn1

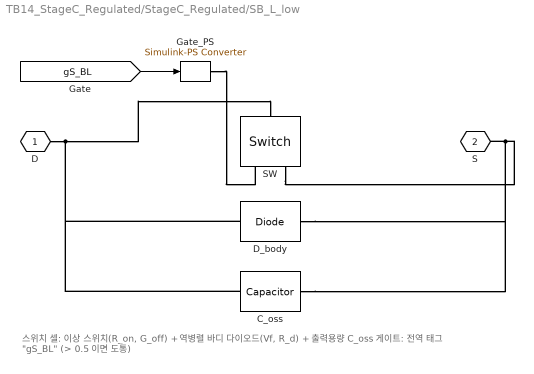
== system TB14_StageC_Regulated/StageC_Regulated/SB_L_low ==
  note: 스위치 셀: 이상 스위치(R_on, G_off) + 역병렬 바디 다이오드(Vf, R_d) + 출력용량 C_oss
      | 게이트: 전역 태그 "gS_BL" (> 0.5 이면 도통)
  C_oss : fl_lib/Electrical/Electrical Elements/Capacitor  c=Coss F  r=1e-6 Ohm  g=0 1/Ohm  i_specify=off  i_priority=None  i=0 A  i_nominal_specify=off  i_nominal_value=1  i_nominal_unit=A  v_specify=off  v_priority=None  v=0 V  v_nominal_specify=off  v_nominal_value=1  v_nominal_unit=V  vc_specify=off  vc_priority=High  vc=0 V  vc_nominal_specify=off  vc_nominal_value=1  vc_nominal_unit=V
  D_body : fl_lib/Electrical/Electrical Elements/Diode  Vf=Vf V  Ron=Rd Ohm  Goff=Goffd 1/Ohm  i_specify=off  i_priority=None  i=0 A  i_nominal_specify=off  i_nominal_value=1  i_nominal_unit=A  v_specify=off  v_priority=None  v=0 V  v_nominal_specify=off  v_nominal_value=1  v_nominal_unit=V
  Gate_PS : nesl_utility/Simulink-PS Converter  PhysicalDomain=network_engine_domain  SubClassName=ps_input  LeftPortType=input  RightPortType=output  PseudoPeriodic=off  Frequencies=[]  NoiseDistribution=none  NoiseParameters=[]  Unit=1  AffineConversion=off  FilteringAndDerivatives=zero  SimscapeFilterOrder=1  InputFilterTimeConstant=0.001  UdotUserProvided=0
  SW : fl_lib/Electrical/Electrical Elements/Switch  R_closed=Ron Ohm  G_open=Goff 1/Ohm  Threshold=0.5  i_specify=off  i_priority=None  i=0 A  i_nominal_specify=off  i_nominal_value=1  i_nominal_unit=A  v_specify=off  v_priority=None  v=0 V  v_nominal_specify=off  v_nominal_value=1  v_nominal_unit=V
  D : PMIOPort  Side=Left
  S : PMIOPort  Port=2  Side=Right
  wires:
  [gS_BL] -> Gate_PS/1
  connections:
  Gate_PS/RConn1 -- SW/RConn1
  SW/LConn1 -- D/RConn1 -- D_body/RConn1 -- C_oss/LConn1
  SW/RConn2 -- D_body/LConn1 -- S/RConn1 -- C_oss/RConn1

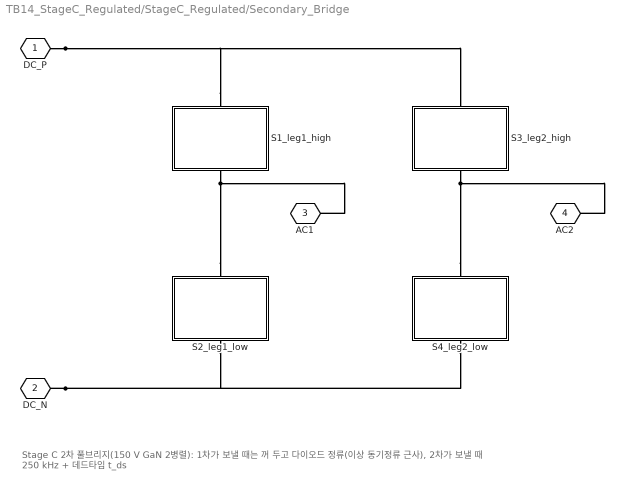
== system TB14_StageC_Regulated/StageC_Regulated/Secondary_Bridge ==
  note: Stage C 2차 풀브리지(150 V GaN 2병렬): 1차가 보낼 때는 꺼 두고 다이오드 정류(이상 동기정류 근사), 2차가 보낼 때 250 kHz + 데드타임 t_ds
  S1_leg1_high : Subsystem  mask(PRISM-Hub switch cell){Ron=TB.CS.Ron, Goff=TB.CS.Goff, Vf=TB.CS.Vf, Rd=TB.CS.Rd, Goffd=TB.CS.Goffd, Coss=TB.CS.Coss}
      mask prompts: Ron "도통 저항 R_on [Ohm]"; Goff "차단 컨덕턴스 G_off [S]"; Vf "다이오드 순방향 전압 Vf [V]"; Rd "다이오드 도통 저항 R_d [Ohm]"; Goffd "다이오드 차단 컨덕턴스 [S]"; Coss "출력용량 C_oss [F]"
      mask help: 전력 반도체 스위치 셀 S1_leg1_high. 게이트 태그 gC_S1.
      settings: AttributesFormatString=gate: gC_S1
      mask Display:
      | plot([0.50 0.50 ],[0.95 0.65 ],[0.50 0.74 ],[0.65 0.35 ],[0.50 0.50 ],[0.35 0.05 ]);
      | plot([0.50 0.20 0.20 ],[0.80 0.80 0.58 ],[0.20 0.20 0.50 ],[0.42 0.20 0.20 ]);
      | plot([0.20 0.10 0.30 0.20 ],[0.58 0.42 0.42 0.58 ],[0.10 0.30 ],[0.58 0.58 ]);
      | port_label('LConn',1,'D');
      | port_label('RConn',1,'S');
  S2_leg1_low : Subsystem  mask(PRISM-Hub switch cell){Ron=TB.CS.Ron, Goff=TB.CS.Goff, Vf=TB.CS.Vf, Rd=TB.CS.Rd, Goffd=TB.CS.Goffd, Coss=TB.CS.Coss}
      mask prompts: Ron "도통 저항 R_on [Ohm]"; Goff "차단 컨덕턴스 G_off [S]"; Vf "다이오드 순방향 전압 Vf [V]"; Rd "다이오드 도통 저항 R_d [Ohm]"; Goffd "다이오드 차단 컨덕턴스 [S]"; Coss "출력용량 C_oss [F]"
      mask help: 전력 반도체 스위치 셀 S2_leg1_low. 게이트 태그 gC_S2.
      settings: AttributesFormatString=gate: gC_S2
      mask Display:
      | plot([0.50 0.50 ],[0.95 0.65 ],[0.50 0.74 ],[0.65 0.35 ],[0.50 0.50 ],[0.35 0.05 ]);
      | plot([0.50 0.20 0.20 ],[0.80 0.80 0.58 ],[0.20 0.20 0.50 ],[0.42 0.20 0.20 ]);
      | plot([0.20 0.10 0.30 0.20 ],[0.58 0.42 0.42 0.58 ],[0.10 0.30 ],[0.58 0.58 ]);
      | port_label('LConn',1,'D');
      | port_label('RConn',1,'S');
  S3_leg2_high : Subsystem  mask(PRISM-Hub switch cell){Ron=TB.CS.Ron, Goff=TB.CS.Goff, Vf=TB.CS.Vf, Rd=TB.CS.Rd, Goffd=TB.CS.Goffd, Coss=TB.CS.Coss}
      mask prompts: Ron "도통 저항 R_on [Ohm]"; Goff "차단 컨덕턴스 G_off [S]"; Vf "다이오드 순방향 전압 Vf [V]"; Rd "다이오드 도통 저항 R_d [Ohm]"; Goffd "다이오드 차단 컨덕턴스 [S]"; Coss "출력용량 C_oss [F]"
      mask help: 전력 반도체 스위치 셀 S3_leg2_high. 게이트 태그 gC_S3.
      settings: AttributesFormatString=gate: gC_S3
      mask Display:
      | plot([0.50 0.50 ],[0.95 0.65 ],[0.50 0.74 ],[0.65 0.35 ],[0.50 0.50 ],[0.35 0.05 ]);
      | plot([0.50 0.20 0.20 ],[0.80 0.80 0.58 ],[0.20 0.20 0.50 ],[0.42 0.20 0.20 ]);
      | plot([0.20 0.10 0.30 0.20 ],[0.58 0.42 0.42 0.58 ],[0.10 0.30 ],[0.58 0.58 ]);
      | port_label('LConn',1,'D');
      | port_label('RConn',1,'S');
  S4_leg2_low : Subsystem  mask(PRISM-Hub switch cell){Ron=TB.CS.Ron, Goff=TB.CS.Goff, Vf=TB.CS.Vf, Rd=TB.CS.Rd, Goffd=TB.CS.Goffd, Coss=TB.CS.Coss}
      mask prompts: Ron "도통 저항 R_on [Ohm]"; Goff "차단 컨덕턴스 G_off [S]"; Vf "다이오드 순방향 전압 Vf [V]"; Rd "다이오드 도통 저항 R_d [Ohm]"; Goffd "다이오드 차단 컨덕턴스 [S]"; Coss "출력용량 C_oss [F]"
      mask help: 전력 반도체 스위치 셀 S4_leg2_low. 게이트 태그 gC_S4.
      settings: AttributesFormatString=gate: gC_S4
      mask Display:
      | plot([0.50 0.50 ],[0.95 0.65 ],[0.50 0.74 ],[0.65 0.35 ],[0.50 0.50 ],[0.35 0.05 ]);
      | plot([0.50 0.20 0.20 ],[0.80 0.80 0.58 ],[0.20 0.20 0.50 ],[0.42 0.20 0.20 ]);
      | plot([0.20 0.10 0.30 0.20 ],[0.58 0.42 0.42 0.58 ],[0.10 0.30 ],[0.58 0.58 ]);
      | port_label('LConn',1,'D');
      | port_label('RConn',1,'S');
  DC_P : PMIOPort  Side=Left
  DC_N : PMIOPort  Port=2  Side=Left
  AC1 : PMIOPort  Port=3  Side=Right
  AC2 : PMIOPort  Port=4  Side=Right
  connections:
  S1_leg1_high/LConn1 -- DC_P/RConn1 -- S3_leg2_high/LConn1
  S2_leg1_low/LConn1 -- S1_leg1_high/RConn1 -- AC1/RConn1
  S4_leg2_low/LConn1 -- S3_leg2_high/RConn1 -- AC2/RConn1
  DC_N/RConn1 -- S2_leg1_low/RConn1 -- S4_leg2_low/RConn1

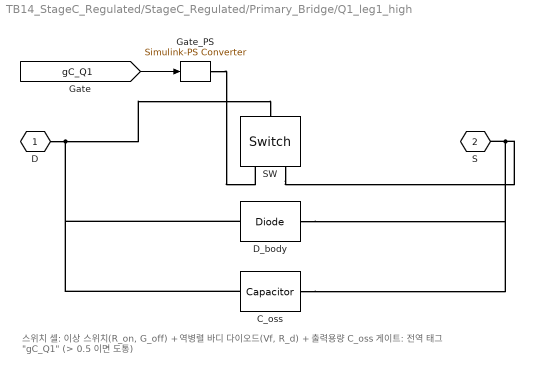
== system TB14_StageC_Regulated/StageC_Regulated/Primary_Bridge/Q1_leg1_high ==
  note: 스위치 셀: 이상 스위치(R_on, G_off) + 역병렬 바디 다이오드(Vf, R_d) + 출력용량 C_oss
      | 게이트: 전역 태그 "gC_Q1" (> 0.5 이면 도통)
  C_oss : fl_lib/Electrical/Electrical Elements/Capacitor  c=Coss F  r=1e-6 Ohm  g=0 1/Ohm  i_specify=off  i_priority=None  i=0 A  i_nominal_specify=off  i_nominal_value=1  i_nominal_unit=A  v_specify=off  v_priority=None  v=0 V  v_nominal_specify=off  v_nominal_value=1  v_nominal_unit=V  vc_specify=off  vc_priority=High  vc=0 V  vc_nominal_specify=off  vc_nominal_value=1  vc_nominal_unit=V
  D_body : fl_lib/Electrical/Electrical Elements/Diode  Vf=Vf V  Ron=Rd Ohm  Goff=Goffd 1/Ohm  i_specify=off  i_priority=None  i=0 A  i_nominal_specify=off  i_nominal_value=1  i_nominal_unit=A  v_specify=off  v_priority=None  v=0 V  v_nominal_specify=off  v_nominal_value=1  v_nominal_unit=V
  Gate_PS : nesl_utility/Simulink-PS Converter  PhysicalDomain=network_engine_domain  SubClassName=ps_input  LeftPortType=input  RightPortType=output  PseudoPeriodic=off  Frequencies=[]  NoiseDistribution=none  NoiseParameters=[]  Unit=1  AffineConversion=off  FilteringAndDerivatives=zero  SimscapeFilterOrder=1  InputFilterTimeConstant=0.001  UdotUserProvided=0
  SW : fl_lib/Electrical/Electrical Elements/Switch  R_closed=Ron Ohm  G_open=Goff 1/Ohm  Threshold=0.5  i_specify=off  i_priority=None  i=0 A  i_nominal_specify=off  i_nominal_value=1  i_nominal_unit=A  v_specify=off  v_priority=None  v=0 V  v_nominal_specify=off  v_nominal_value=1  v_nominal_unit=V
  D : PMIOPort  Side=Left
  S : PMIOPort  Port=2  Side=Right
  wires:
  [gC_Q1] -> Gate_PS/1
  connections:
  Gate_PS/RConn1 -- SW/RConn1
  SW/LConn1 -- D/RConn1 -- D_body/RConn1 -- C_oss/LConn1
  SW/RConn2 -- D_body/LConn1 -- S/RConn1 -- C_oss/RConn1

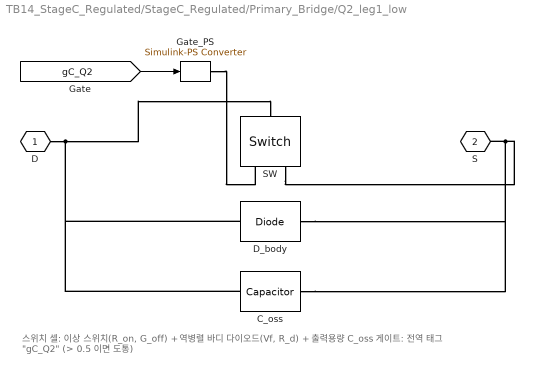
== system TB14_StageC_Regulated/StageC_Regulated/Primary_Bridge/Q2_leg1_low ==
  note: 스위치 셀: 이상 스위치(R_on, G_off) + 역병렬 바디 다이오드(Vf, R_d) + 출력용량 C_oss
      | 게이트: 전역 태그 "gC_Q2" (> 0.5 이면 도통)
  C_oss : fl_lib/Electrical/Electrical Elements/Capacitor  c=Coss F  r=1e-6 Ohm  g=0 1/Ohm  i_specify=off  i_priority=None  i=0 A  i_nominal_specify=off  i_nominal_value=1  i_nominal_unit=A  v_specify=off  v_priority=None  v=0 V  v_nominal_specify=off  v_nominal_value=1  v_nominal_unit=V  vc_specify=off  vc_priority=High  vc=0 V  vc_nominal_specify=off  vc_nominal_value=1  vc_nominal_unit=V
  D_body : fl_lib/Electrical/Electrical Elements/Diode  Vf=Vf V  Ron=Rd Ohm  Goff=Goffd 1/Ohm  i_specify=off  i_priority=None  i=0 A  i_nominal_specify=off  i_nominal_value=1  i_nominal_unit=A  v_specify=off  v_priority=None  v=0 V  v_nominal_specify=off  v_nominal_value=1  v_nominal_unit=V
  Gate_PS : nesl_utility/Simulink-PS Converter  PhysicalDomain=network_engine_domain  SubClassName=ps_input  LeftPortType=input  RightPortType=output  PseudoPeriodic=off  Frequencies=[]  NoiseDistribution=none  NoiseParameters=[]  Unit=1  AffineConversion=off  FilteringAndDerivatives=zero  SimscapeFilterOrder=1  InputFilterTimeConstant=0.001  UdotUserProvided=0
  SW : fl_lib/Electrical/Electrical Elements/Switch  R_closed=Ron Ohm  G_open=Goff 1/Ohm  Threshold=0.5  i_specify=off  i_priority=None  i=0 A  i_nominal_specify=off  i_nominal_value=1  i_nominal_unit=A  v_specify=off  v_priority=None  v=0 V  v_nominal_specify=off  v_nominal_value=1  v_nominal_unit=V
  D : PMIOPort  Side=Left
  S : PMIOPort  Port=2  Side=Right
  wires:
  [gC_Q2] -> Gate_PS/1
  connections:
  Gate_PS/RConn1 -- SW/RConn1
  SW/LConn1 -- D/RConn1 -- D_body/RConn1 -- C_oss/LConn1
  SW/RConn2 -- D_body/LConn1 -- S/RConn1 -- C_oss/RConn1

== system TB14_StageC_Regulated/StageC_Regulated/Primary_Bridge/Q3_leg2_high ==
  note: 스위치 셀: 이상 스위치(R_on, G_off) + 역병렬 바디 다이오드(Vf, R_d) + 출력용량 C_oss
      | 게이트: 전역 태그 "gC_Q3" (> 0.5 이면 도통)
  C_oss : fl_lib/Electrical/Electrical Elements/Capacitor  c=Coss F  r=1e-6 Ohm  g=0 1/Ohm  i_specify=off  i_priority=None  i=0 A  i_nominal_specify=off  i_nominal_value=1  i_nominal_unit=A  v_specify=off  v_priority=None  v=0 V  v_nominal_specify=off  v_nominal_value=1  v_nominal_unit=V  vc_specify=off  vc_priority=High  vc=0 V  vc_nominal_specify=off  vc_nominal_value=1  vc_nominal_unit=V
  D_body : fl_lib/Electrical/Electrical Elements/Diode  Vf=Vf V  Ron=Rd Ohm  Goff=Goffd 1/Ohm  i_specify=off  i_priority=None  i=0 A  i_nominal_specify=off  i_nominal_value=1  i_nominal_unit=A  v_specify=off  v_priority=None  v=0 V  v_nominal_specify=off  v_nominal_value=1  v_nominal_unit=V
  Gate_PS : nesl_utility/Simulink-PS Converter  PhysicalDomain=network_engine_domain  SubClassName=ps_input  LeftPortType=input  RightPortType=output  PseudoPeriodic=off  Frequencies=[]  NoiseDistribution=none  NoiseParameters=[]  Unit=1  AffineConversion=off  FilteringAndDerivatives=zero  SimscapeFilterOrder=1  InputFilterTimeConstant=0.001  UdotUserProvided=0
  SW : fl_lib/Electrical/Electrical Elements/Switch  R_closed=Ron Ohm  G_open=Goff 1/Ohm  Threshold=0.5  i_specify=off  i_priority=None  i=0 A  i_nominal_specify=off  i_nominal_value=1  i_nominal_unit=A  v_specify=off  v_priority=None  v=0 V  v_nominal_specify=off  v_nominal_value=1  v_nominal_unit=V
  D : PMIOPort  Side=Left
  S : PMIOPort  Port=2  Side=Right
  wires:
  [gC_Q3] -> Gate_PS/1
  connections:
  Gate_PS/RConn1 -- SW/RConn1
  SW/LConn1 -- D/RConn1 -- D_body/RConn1 -- C_oss/LConn1
  SW/RConn2 -- D_body/LConn1 -- S/RConn1 -- C_oss/RConn1

== system TB14_StageC_Regulated/StageC_Regulated/Primary_Bridge/Q4_leg2_low ==
  note: 스위치 셀: 이상 스위치(R_on, G_off) + 역병렬 바디 다이오드(Vf, R_d) + 출력용량 C_oss
      | 게이트: 전역 태그 "gC_Q4" (> 0.5 이면 도통)
  C_oss : fl_lib/Electrical/Electrical Elements/Capacitor  c=Coss F  r=1e-6 Ohm  g=0 1/Ohm  i_specify=off  i_priority=None  i=0 A  i_nominal_specify=off  i_nominal_value=1  i_nominal_unit=A  v_specify=off  v_priority=None  v=0 V  v_nominal_specify=off  v_nominal_value=1  v_nominal_unit=V  vc_specify=off  vc_priority=High  vc=0 V  vc_nominal_specify=off  vc_nominal_value=1  vc_nominal_unit=V
  D_body : fl_lib/Electrical/Electrical Elements/Diode  Vf=Vf V  Ron=Rd Ohm  Goff=Goffd 1/Ohm  i_specify=off  i_priority=None  i=0 A  i_nominal_specify=off  i_nominal_value=1  i_nominal_unit=A  v_specify=off  v_priority=None  v=0 V  v_nominal_specify=off  v_nominal_value=1  v_nominal_unit=V
  Gate_PS : nesl_utility/Simulink-PS Converter  PhysicalDomain=network_engine_domain  SubClassName=ps_input  LeftPortType=input  RightPortType=output  PseudoPeriodic=off  Frequencies=[]  NoiseDistribution=none  NoiseParameters=[]  Unit=1  AffineConversion=off  FilteringAndDerivatives=zero  SimscapeFilterOrder=1  InputFilterTimeConstant=0.001  UdotUserProvided=0
  SW : fl_lib/Electrical/Electrical Elements/Switch  R_closed=Ron Ohm  G_open=Goff 1/Ohm  Threshold=0.5  i_specify=off  i_priority=None  i=0 A  i_nominal_specify=off  i_nominal_value=1  i_nominal_unit=A  v_specify=off  v_priority=None  v=0 V  v_nominal_specify=off  v_nominal_value=1  v_nominal_unit=V
  D : PMIOPort  Side=Left
  S : PMIOPort  Port=2  Side=Right
  wires:
  [gC_Q4] -> Gate_PS/1
  connections:
  Gate_PS/RConn1 -- SW/RConn1
  SW/LConn1 -- D/RConn1 -- D_body/RConn1 -- C_oss/LConn1
  SW/RConn2 -- D_body/LConn1 -- S/RConn1 -- C_oss/RConn1

== system TB14_StageC_Regulated/StageC_Regulated/Secondary_Bridge/S1_leg1_high ==
  note: 스위치 셀: 이상 스위치(R_on, G_off) + 역병렬 바디 다이오드(Vf, R_d) + 출력용량 C_oss
      | 게이트: 전역 태그 "gC_S1" (> 0.5 이면 도통)
  C_oss : fl_lib/Electrical/Electrical Elements/Capacitor  c=Coss F  r=1e-6 Ohm  g=0 1/Ohm  i_specify=off  i_priority=None  i=0 A  i_nominal_specify=off  i_nominal_value=1  i_nominal_unit=A  v_specify=off  v_priority=None  v=0 V  v_nominal_specify=off  v_nominal_value=1  v_nominal_unit=V  vc_specify=off  vc_priority=High  vc=0 V  vc_nominal_specify=off  vc_nominal_value=1  vc_nominal_unit=V
  D_body : fl_lib/Electrical/Electrical Elements/Diode  Vf=Vf V  Ron=Rd Ohm  Goff=Goffd 1/Ohm  i_specify=off  i_priority=None  i=0 A  i_nominal_specify=off  i_nominal_value=1  i_nominal_unit=A  v_specify=off  v_priority=None  v=0 V  v_nominal_specify=off  v_nominal_value=1  v_nominal_unit=V
  Gate_PS : nesl_utility/Simulink-PS Converter  PhysicalDomain=network_engine_domain  SubClassName=ps_input  LeftPortType=input  RightPortType=output  PseudoPeriodic=off  Frequencies=[]  NoiseDistribution=none  NoiseParameters=[]  Unit=1  AffineConversion=off  FilteringAndDerivatives=zero  SimscapeFilterOrder=1  InputFilterTimeConstant=0.001  UdotUserProvided=0
  SW : fl_lib/Electrical/Electrical Elements/Switch  R_closed=Ron Ohm  G_open=Goff 1/Ohm  Threshold=0.5  i_specify=off  i_priority=None  i=0 A  i_nominal_specify=off  i_nominal_value=1  i_nominal_unit=A  v_specify=off  v_priority=None  v=0 V  v_nominal_specify=off  v_nominal_value=1  v_nominal_unit=V
  D : PMIOPort  Side=Left
  S : PMIOPort  Port=2  Side=Right
  wires:
  [gC_S1] -> Gate_PS/1
  connections:
  Gate_PS/RConn1 -- SW/RConn1
  SW/LConn1 -- D/RConn1 -- D_body/RConn1 -- C_oss/LConn1
  SW/RConn2 -- D_body/LConn1 -- S/RConn1 -- C_oss/RConn1

== system TB14_StageC_Regulated/StageC_Regulated/Secondary_Bridge/S2_leg1_low ==
  note: 스위치 셀: 이상 스위치(R_on, G_off) + 역병렬 바디 다이오드(Vf, R_d) + 출력용량 C_oss
      | 게이트: 전역 태그 "gC_S2" (> 0.5 이면 도통)
  C_oss : fl_lib/Electrical/Electrical Elements/Capacitor  c=Coss F  r=1e-6 Ohm  g=0 1/Ohm  i_specify=off  i_priority=None  i=0 A  i_nominal_specify=off  i_nominal_value=1  i_nominal_unit=A  v_specify=off  v_priority=None  v=0 V  v_nominal_specify=off  v_nominal_value=1  v_nominal_unit=V  vc_specify=off  vc_priority=High  vc=0 V  vc_nominal_specify=off  vc_nominal_value=1  vc_nominal_unit=V
  D_body : fl_lib/Electrical/Electrical Elements/Diode  Vf=Vf V  Ron=Rd Ohm  Goff=Goffd 1/Ohm  i_specify=off  i_priority=None  i=0 A  i_nominal_specify=off  i_nominal_value=1  i_nominal_unit=A  v_specify=off  v_priority=None  v=0 V  v_nominal_specify=off  v_nominal_value=1  v_nominal_unit=V
  Gate_PS : nesl_utility/Simulink-PS Converter  PhysicalDomain=network_engine_domain  SubClassName=ps_input  LeftPortType=input  RightPortType=output  PseudoPeriodic=off  Frequencies=[]  NoiseDistribution=none  NoiseParameters=[]  Unit=1  AffineConversion=off  FilteringAndDerivatives=zero  SimscapeFilterOrder=1  InputFilterTimeConstant=0.001  UdotUserProvided=0
  SW : fl_lib/Electrical/Electrical Elements/Switch  R_closed=Ron Ohm  G_open=Goff 1/Ohm  Threshold=0.5  i_specify=off  i_priority=None  i=0 A  i_nominal_specify=off  i_nominal_value=1  i_nominal_unit=A  v_specify=off  v_priority=None  v=0 V  v_nominal_specify=off  v_nominal_value=1  v_nominal_unit=V
  D : PMIOPort  Side=Left
  S : PMIOPort  Port=2  Side=Right
  wires:
  [gC_S2] -> Gate_PS/1
  connections:
  Gate_PS/RConn1 -- SW/RConn1
  SW/LConn1 -- D/RConn1 -- D_body/RConn1 -- C_oss/LConn1
  SW/RConn2 -- D_body/LConn1 -- S/RConn1 -- C_oss/RConn1

== system TB14_StageC_Regulated/StageC_Regulated/Secondary_Bridge/S3_leg2_high ==
  note: 스위치 셀: 이상 스위치(R_on, G_off) + 역병렬 바디 다이오드(Vf, R_d) + 출력용량 C_oss
      | 게이트: 전역 태그 "gC_S3" (> 0.5 이면 도통)
  C_oss : fl_lib/Electrical/Electrical Elements/Capacitor  c=Coss F  r=1e-6 Ohm  g=0 1/Ohm  i_specify=off  i_priority=None  i=0 A  i_nominal_specify=off  i_nominal_value=1  i_nominal_unit=A  v_specify=off  v_priority=None  v=0 V  v_nominal_specify=off  v_nominal_value=1  v_nominal_unit=V  vc_specify=off  vc_priority=High  vc=0 V  vc_nominal_specify=off  vc_nominal_value=1  vc_nominal_unit=V
  D_body : fl_lib/Electrical/Electrical Elements/Diode  Vf=Vf V  Ron=Rd Ohm  Goff=Goffd 1/Ohm  i_specify=off  i_priority=None  i=0 A  i_nominal_specify=off  i_nominal_value=1  i_nominal_unit=A  v_specify=off  v_priority=None  v=0 V  v_nominal_specify=off  v_nominal_value=1  v_nominal_unit=V
  Gate_PS : nesl_utility/Simulink-PS Converter  PhysicalDomain=network_engine_domain  SubClassName=ps_input  LeftPortType=input  RightPortType=output  PseudoPeriodic=off  Frequencies=[]  NoiseDistribution=none  NoiseParameters=[]  Unit=1  AffineConversion=off  FilteringAndDerivatives=zero  SimscapeFilterOrder=1  InputFilterTimeConstant=0.001  UdotUserProvided=0
  SW : fl_lib/Electrical/Electrical Elements/Switch  R_closed=Ron Ohm  G_open=Goff 1/Ohm  Threshold=0.5  i_specify=off  i_priority=None  i=0 A  i_nominal_specify=off  i_nominal_value=1  i_nominal_unit=A  v_specify=off  v_priority=None  v=0 V  v_nominal_specify=off  v_nominal_value=1  v_nominal_unit=V
  D : PMIOPort  Side=Left
  S : PMIOPort  Port=2  Side=Right
  wires:
  [gC_S3] -> Gate_PS/1
  connections:
  Gate_PS/RConn1 -- SW/RConn1
  SW/LConn1 -- D/RConn1 -- D_body/RConn1 -- C_oss/LConn1
  SW/RConn2 -- D_body/LConn1 -- S/RConn1 -- C_oss/RConn1

== system TB14_StageC_Regulated/StageC_Regulated/Secondary_Bridge/S4_leg2_low ==
  note: 스위치 셀: 이상 스위치(R_on, G_off) + 역병렬 바디 다이오드(Vf, R_d) + 출력용량 C_oss
      | 게이트: 전역 태그 "gC_S4" (> 0.5 이면 도통)
  C_oss : fl_lib/Electrical/Electrical Elements/Capacitor  c=Coss F  r=1e-6 Ohm  g=0 1/Ohm  i_specify=off  i_priority=None  i=0 A  i_nominal_specify=off  i_nominal_value=1  i_nominal_unit=A  v_specify=off  v_priority=None  v=0 V  v_nominal_specify=off  v_nominal_value=1  v_nominal_unit=V  vc_specify=off  vc_priority=High  vc=0 V  vc_nominal_specify=off  vc_nominal_value=1  vc_nominal_unit=V
  D_body : fl_lib/Electrical/Electrical Elements/Diode  Vf=Vf V  Ron=Rd Ohm  Goff=Goffd 1/Ohm  i_specify=off  i_priority=None  i=0 A  i_nominal_specify=off  i_nominal_value=1  i_nominal_unit=A  v_specify=off  v_priority=None  v=0 V  v_nominal_specify=off  v_nominal_value=1  v_nominal_unit=V
  Gate_PS : nesl_utility/Simulink-PS Converter  PhysicalDomain=network_engine_domain  SubClassName=ps_input  LeftPortType=input  RightPortType=output  PseudoPeriodic=off  Frequencies=[]  NoiseDistribution=none  NoiseParameters=[]  Unit=1  AffineConversion=off  FilteringAndDerivatives=zero  SimscapeFilterOrder=1  InputFilterTimeConstant=0.001  UdotUserProvided=0
  SW : fl_lib/Electrical/Electrical Elements/Switch  R_closed=Ron Ohm  G_open=Goff 1/Ohm  Threshold=0.5  i_specify=off  i_priority=None  i=0 A  i_nominal_specify=off  i_nominal_value=1  i_nominal_unit=A  v_specify=off  v_priority=None  v=0 V  v_nominal_specify=off  v_nominal_value=1  v_nominal_unit=V
  D : PMIOPort  Side=Left
  S : PMIOPort  Port=2  Side=Right
  wires:
  [gC_S4] -> Gate_PS/1
  connections:
  Gate_PS/RConn1 -- SW/RConn1
  SW/LConn1 -- D/RConn1 -- D_body/RConn1 -- C_oss/LConn1
  SW/RConn2 -- D_body/LConn1 -- S/RConn1 -- C_oss/RConn1

== matlab function TB14_StageC_Regulated/Test_Conditions/Profile ==
  data: t input; y output; prm input
function y = prism_tb14_profile(t, prm)
%#codegen
%PRISM_TB14_PROFILE  TB14 시험 조건: 버스 전압 지령과 48 V 정전력 부하 전력의 구간 선형 시간 함수(시험 장치, 제어기 아님).
%
%   prm = [t_V(1:4) V(1:4) t_P(1:4) P(1:4)]  (점이 4개보다 적으면 마지막 점을 반복해 채운다)
%   출력 y = [v_bus 지령 [V]; p_load [W]](p_load < 0이면 48 V 쪽 발전원)

tV = prm(1:4); V = prm(5:8); tP = prm(9:12); P = prm(13:16);
y = [pwl(t, tV, V); pwl(t, tP, P)];
end

function v = pwl(t, tt, yy)
v = yy(4);
if t <= tt(1)
    v = yy(1);
    return
end
for k = 2:4
    if t <= tt(k)
        if tt(k) > tt(k-1)
            v = yy(k-1) + (yy(k) - yy(k-1))*(t - tt(k-1))/(tt(k) - tt(k-1));
        else
            v = yy(k);
        end
        return
    end
end
end
